simulink model "MMC_phase_hackathon_consensus_PWM_JABBAR_20260927"  (R2024b)
settings: Solver=FixedStepDiscrete  StartTime=t_init_sim  StopTime=sim_time  FixedStep=Ts  RelTol=1e-3
values from neighbouring files (symbols this model uses):
  a = 1    [script_MMC_phase_hackathon_consensus_PWM_JABBAR_20260927.m]
  C1low1_active = 1    [script_MMC_phase_hackathon_consensus_PWM_JABBAR_20260927.m]
  C2low1_active = 1    [script_MMC_phase_hackathon_consensus_PWM_JABBAR_20260927.m]
  C_bus = 4400e-6    (= 0.0044)    [script_MMC_phase_hackathon_consensus_PWM_JABBAR_20260927.m]
  C_M_extra = C_m-twist_high_side_C    [script_MMC_phase_hackathon_consensus_PWM_JABBAR_20260927.m]
  f0 = 50    [script_MMC_phase_hackathon_consensus_PWM_JABBAR_20260927.m]
  feeder_current_lower_rate_limit = -10    [script_MMC_phase_hackathon_consensus_PWM_JABBAR_20260927.m]    (also in twist_parameters.m = -500)
  feeder_current_tab = [0.328 0.217 0.162 0.132 0.109 0.094 0.083 0.075 0.068 0.062 0.058 0.054 ... (42 elements, 14x3)]    [feeder_current.mat]
  feeder_current_upper_rate_limit = 0.386/(20e-3)    (= 19.3)    [twist_parameters.m]
  is6VExternallySupplied = true    [script_MMC_phase_hackathon_consensus_PWM_JABBAR_20260927.m]
  isFeederJumperOpen = true    [script_MMC_phase_hackathon_consensus_PWM_JABBAR_20260927.m]
  L_arm = 100e-3    (= 0.1)    [script_MMC_phase_hackathon_consensus_PWM_JABBAR_20260927.m]
  m = 1    [script_MMC_phase_hackathon_consensus_PWM_JABBAR_20260927.m]
  power_losses = false    [script_MMC_phase_hackathon_consensus_PWM_JABBAR_20260927.m]
  R = 30    [script_MMC_phase_hackathon_consensus_PWM_JABBAR_20260927.m]
  R_arm = 0.2    [script_MMC_phase_hackathon_consensus_PWM_JABBAR_20260927.m]
  source_V = 0    [script_MMC_phase_hackathon_consensus_PWM_JABBAR_20260927.m]
  time_charge = 0.1    [script_MMC_phase_hackathon_consensus_PWM_JABBAR_20260927.m]
  time_decharge = 1.5    [script_MMC_phase_hackathon_consensus_PWM_JABBAR_20260927.m]
  Ts = 5e-7    (= 5e-07)    [script_MMC_phase_hackathon_consensus_PWM_JABBAR_20260927.m]
  twist_data_acquisition_delay = 50e-9    (= 5e-08)    [script_MMC_phase_hackathon_consensus_PWM_JABBAR_20260927.m]    (also in twist_parameters.m)
  twist_data_sampling_period = 1/twist_freq_data_sampling    (= 5e-05)    [script_MMC_phase_hackathon_consensus_PWM_JABBAR_20260927.m]    (also in twist_parameters.m)
  twist_dead_time = 200e-9    (= 2e-07)    [twist_parameters.m]
  twist_freq_switching = 200e3    (= 200000)    [twist_parameters.m]
  twist_high_side_adc_R = 1/(1/2e6 + 1/2e6 + 1/(330e3+5.6e3))    (= 251272.836178)    [twist_parameters.m]
  twist_high_side_C = 33e-6*4 + 4.7e-6*12    (= 0.0001884)    [twist_parameters.m]
  twist_high_side_feeder_R = 47e3+4.7e3    (= 51700)    [twist_parameters.m]
  twist_high_side_rC = 0.1    [twist_parameters.m]
  twist_low_side_adc_R = 150e3+470    (= 150470)    [twist_parameters.m]
  twist_low_side_C_ceramic = 3*4.7e-6    (= 1.41e-05)    [twist_parameters.m]
  twist_low_side_C_electrolytic = 47e-6    (= 4.7e-05)    [twist_parameters.m]
  twist_low_side_L = 33e-6    (= 3.3e-05)    [twist_parameters.m]
  twist_low_side_rC = 700e-3    (= 0.7)    [twist_parameters.m]
  twist_low_side_rL = 20e-3    (= 0.02)    [twist_parameters.m]
  twist_R_VCC = (tau_VCC/twist_high_side_C  - twist_high_side_rC)/(1-(tau_VCC/twist_high_side_C - twist_high_side_rC)/R_parallel)    (= 1110.74997822)    [twist_parameters.m]
  VDC = 48    [script_MMC_phase_hackathon_consensus_PWM_JABBAR_20260927.m]
undefined symbols (not defined in the file or in its folder): C_SM, feeder_current, gcbh, sps_rtmsupport, twist_low_side_lC
libraries: spsSeriesRLCBranchLib x135, spsTriangleGeneratorLib x60, spsMosfetLib x60, spsCurrentMeasurementLib x43, spsVoltageMeasurementLib x35, spsControlledCurrentSourceLib x30, spsDiodeLib x22, spsIdealSwitchLib x20, spsControlledVoltageSourceLib x1, spsGroundLib x1, spspowerguiLib x1
(part 1 of 19)
settings Model: Creator=ana  LastModifiedBy=ana

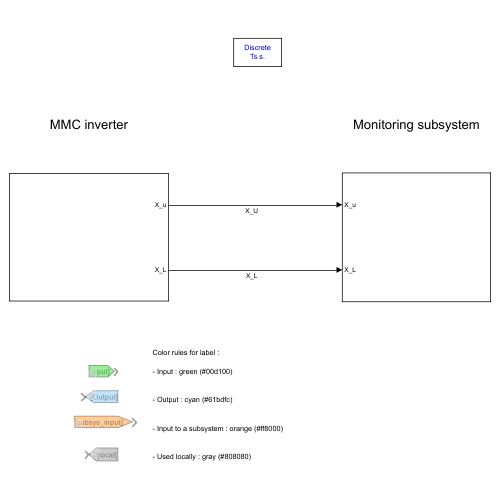
[thumbnail: Simulink's stored preview of the top-level diagram]
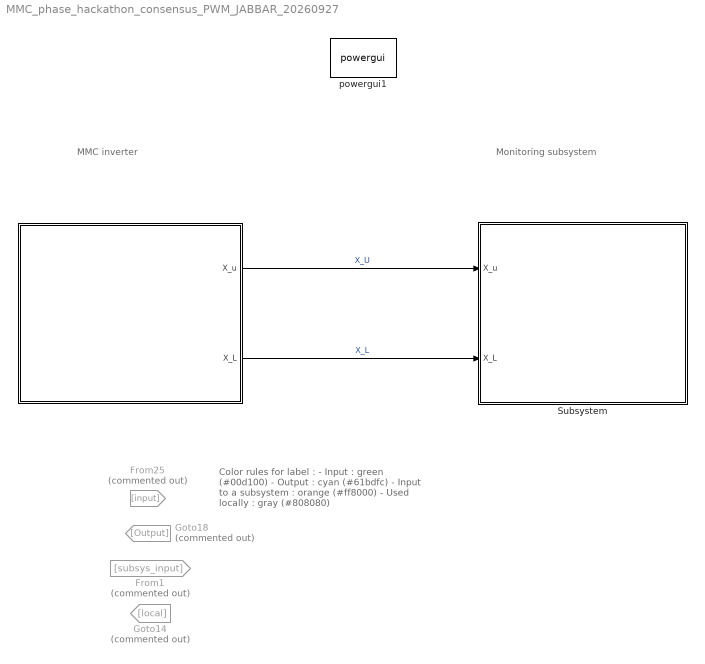
== system MMC_phase_hackathon_consensus_PWM_JABBAR_20260927 ==
  note: Color rules for label :
      |
      | - Input : green (#00d100)
      |
      |
      | - Output : cyan (#61bdfc)
      |
      |
      | - Input to a subsystem : orange (#ff8000)
      |
      |
      | - Used locally : gray (#808080)
  note: MMC inverter
  note: Monitoring subsystem
  " " : Subsystem
  From1 : From  Commented=on  GotoTag=subsys_input
  From25 : From  Commented=on  GotoTag=input
  Goto14 : Goto  Commented=on  GotoTag=local
  Goto18 : Goto  Commented=on  GotoTag=Output
  Subsystem : Subsystem
  powergui1 : spspowerguiLib/powergui  Priority=1  SimulationMode=Discrete  SampleTime=Ts  frequency=60  Iterations=50  frequencyindice=0  Pbase=100e6  ErrMax=1e-4  UnitsV=V  UnitsW=W  buscounter=0  FunctionMessages=off  echomessages=off  EnableUseOfTLC=off  CurrentSourceSwitches=off  DisableSnubberDevices=off  DisableRonSwitches=off  DisableVfSwitches=off  DisplayEquations=off  AutomaticDiscreteSolvers=off  SolverType=Backward Euler  Interpol=off  ExternalGateDelay=off  methode=off  Ts=0  x0status=blocks  SPID=off  SwTol=0  HookPort=off  NonlinearTolerance=1e-4  nMaxIteration=100  ContinueOnMaxIteration=off  RestoreLinks=warning  ResistiveCurrentMeasurement=off  Frange=[0:2:500]  Ylog=off  Xlog=on  ShowGrid=off  save=off  variable=ZData  structure=0  ZoomFFT=off  StartTime=0.0  cycles=1  DisplayStyle=1  fundamental=60  FreqAxis=off  MaxFrequency=1000  frequencyindicesteady=1  RmsSteady=1  display=off
  wires:
  " "/1(X_u) -> Subsystem/1(X_u)  "X_U"
  " "/2(X_L) -> Subsystem/2(X_L)  "X_L"

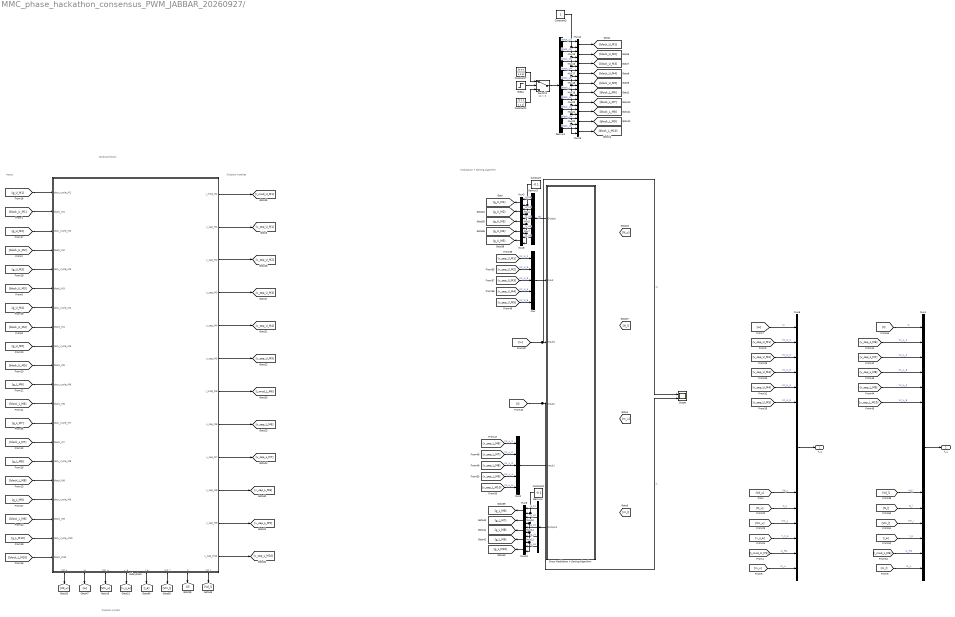
== system MMC_phase_hackathon_consensus_PWM_JABBAR_20260927/  ==
  note: Inputs
  note: Modulation + Sorting Algorithm
  note: Outputs modules
  note: Outputs system
  note: Hardware block
  Constant : Constant  Value=-0.1
  Constant1 : Constant  Value=-0.1
  Constant2 : Constant  Value=[1 1 1 1 1 1 1 1 1 1]
  Constant3 : Constant
  Constant7 : Constant  Value=[0 0 0 0 0 0 0 0 0 0]
  Demux1 : Demux  Outputs=10
  Demux3 : Demux  Outputs=5
  Demux4 : Demux  Outputs=5
  Mux : Mux  Inputs=5
  Mux1 : Mux  Inputs=17
  Mux{3..5,7..23} (20 alike) : Mux  Inputs=2
  Mux2 : Mux  Inputs=5
  Mux6 : Mux  Inputs=17
  Scope : Scope  NumInputPorts=2
  Sinus Modulation + Sorting Algorithm : Subsystem
      settings: PortSchema="{\"entries\":[{\"content\":{\"sides\":[{\"content\":{\"connectorIds\":[\"Out1\",\"In1\",\"In2\",\"In3\",\"In4\",\"Out2\"]},\"type\":\"ConnectorPlacement.EquallySpacedRectSide\",\"uuid\":\"ad8c3084-d308-4367-9563-bcedaf510cf0\"},{\"content\":{\"side\":\"RIGHT\"},\"type\":\"ConnectorPlacement.EquallySpacedRectSide\",\"uuid\":\"bc60d766-efa5-4acc-9a9d-e305ac7836ae\"},{\"content\":{\"side\":\"TOP\"},\"type\":\"ConnectorPlacement.EquallySpacedRectSide\",\"uuid\":\"8fba04a6-3f78-400c-9de2-20d6df686ca2\"}]},\"type\":\"ConnectorPlacement.EquallySpacedConnector\",\"uuid\":\"e4a9f561-cf27-428b-9d42-5aa201811d00\"}],\"packageUris\":[\"http://schema.mathworks.com/mf0/Connector/R2020b\"],\"version\":\"1.0\"}"
  Step1 : Step  Time=time_charge  SampleTime=Ts
  Subsystem : Subsystem
      settings: PortSchema="{\"entries\":[{\"content\":{\"sides\":[{\"content\":{\"connectorIds\":[\"In1\",\"In2\",\"In3\",\"In4\",\"In5\",\"In6\",\"In7\",\"In8\",\"In9\",\"In10\",\"In11\",\"In12\",\"In13\",\"In14\",\"In15\",\"In16\",\"In17\",\"In18\",\"In19\",\"In20\"]},\"type\":\"ConnectorPlacement.EquallySpacedRectSide\",\"uuid\":\"46d0b6b2-241e-4eaa-b5f4-7cb03ad6e4f0\"},{\"content\":{\"connectorIds\":[\"Out1\",\"Out2\",\"Out3\",\"Out4\",\"Out5\",\"Out6\",\"Out7\",\"Out8\",\"Out9\",\"Out10\",\"Out11\",\"Out12\"],\"side\":\"RIGHT\"},\"type\":\"ConnectorPlacement.EquallySpacedRectSide\",\"uuid\":\"f0391c40-5bbd-42ea-8549-0acba96c1793\"},{\"content\":{\"side\":\"TOP\"},\"type\":\"ConnectorPlacement.EquallySpacedRectSide\",\"uuid\":\"1ede63b4-6869-46b3-8b67-84e7db18bcff\"},{\"content\":{\"connectorIds\":[\"Out13\",\"Out14\",\"Out15\",\"Out16\",\"Out17\",\"Out18\",\"Out19\",\"Out20\"],\"side\":\"BOTTOM\"},\"type\":\"ConnectorPlacement.EquallySpacedRectSide\",\"uuid\":\"c0e3b199-6126-45b0-9783-8fc4162e2280\"}]},\"type\":\"ConnectorPlacement.EquallySpacedConnector\",\"uuid\":\"8bedc799-aa9e-49e4-9c41-8dbcca404e51\"}],\"packageUris\":[\"http://schema.mathworks.com/mf0/Connector/R2020b\"],\"version\":\"1.0\"}"
  Switch1 : Switch  Criteria=u2 > Threshold  SaturateOnIntegerOverflow=off  InputSameDT=off
  X_u : Outport
  X_L : Outport  Port=2
  wires:
  Mux6/1 -> X_u/1
  [iu] -> Mux6/1  "Iu"
  [Vd_u] -> Mux6/12  "Vd_u"
  ? -> [N_u]  "N_u"
  [N_u] -> Mux6/13  "N_u"
  [Vm_u] -> Mux6/14  "Vm_u"
  [v_s_a] -> Mux6/15  "V_s_a"
  Step1/1 -> Switch1/2
  Switch1/1 -> Demux1/1
  Constant7/1 -> Switch1/1
  Constant2/1 -> Switch1/3
  [i_mod_U_M1] -> Mux6/16  "Iu_M1"
  ? -> [N_l]  "N_l"
  [il] -> Mux1/1  "iL"
  Mux1/1 -> X_L/1
  [i_mod_L_M6] -> Mux1/16  "iL_M1"
  [Vd_l] -> Mux1/12  "Vd_l"
  [Vm_l] -> Mux1/14  "Vm_l"
  [N_l] -> Mux1/13  "N_l"
  [i_a] -> Mux1/15  "I_a"
  [v_cap_U_M1] -> Mux6/2  "Vc_U_1"
  [v_cap_U_M2] -> Mux6/3  "Vc_U_2"
  [v_cap_U_M3] -> Mux6/4  "Vc_U_3"
  [v_cap_U_M4] -> Mux6/5  "Vc_U_4"
  [v_cap_U_M5] -> Mux6/6  "Vc_U_5"
  ? -> Mux6/7  "Vm_U_1"
  ? -> Mux6/8  "Vm_U_2"
  ? -> Mux6/9  "Vm_U_3"
  ? -> Mux6/10  "Vm_U_4"
  ? -> Mux6/11  "Vm_U_5"
  [v_cap_L_M6] -> Mux1/2  "Vc_L_1"
  [v_cap_L_M7] -> Mux1/3  "Vc_L_2"
  [v_cap_L_M8] -> Mux1/4  "Vc_L_3"
  [v_cap_L_M9] -> Mux1/5  "Vc_L_4"
  [v_cap_L_M10] -> Mux1/6  "Vc_L_5"
  ? -> Mux1/7  "Vm_L_1"
  ? -> Mux1/8  "Vm_L_2"
  ? -> Mux1/9  "Vm_L_3"
  ? -> Mux1/10  "Vm_L_4"
  ? -> Mux1/11  "Vm_L_5"
  ? -> [m_u]  "m_u"
  ? -> [m_l]  "m_l"
  [m_u] -> Mux6/17  "m_u"
  [m_l] -> Mux1/17  "m_L"
  Sinus Modulation + Sorting Algorithm/1(Output) -> Demux3/1  "gU"
  Mux/1 -> Sinus Modulation + Sorting Algorithm/1(Input)
  [v_cap_U_M1] -> Mux/1  "Vc_U_1"
  [v_cap_U_M2] -> Mux/2  "Vc_U_2"
  [v_cap_U_M3] -> Mux/3  "Vc_U_3"
  [v_cap_U_M4] -> Mux/4  "Vc_U_4"
  [v_cap_U_M5] -> Mux/5  "Vc_U_5"
  [v_cap_L_M6] -> Mux2/1  "Vc_L_1"
  [v_cap_L_M7] -> Mux2/2  "Vc_L_2"
  [v_cap_L_M8] -> Mux2/3  "Vc_L_3"
  [v_cap_L_M9] -> Mux2/4  "Vc_L_4"
  [v_cap_L_M10] -> Mux2/5  "Vc_L_5"
  Mux3/1 -> [g_U_M1]
  Mux8/1 -> [g_U_M5]
  Mux7/1 -> [g_U_M4]
  Mux5/1 -> [g_U_M3]
  Mux4/1 -> [g_U_M2]
  Demux3/1 -> Mux3/1  "g_U1"
  Demux3/2 -> Mux4/1  "g_U2"
  Demux3/3 -> Mux5/1  "g_U3"
  Demux3/4 -> Mux7/1  "g_U4"
  Demux3/5 -> Mux8/1  "g_U5"
  Constant/1 -> Mux8/2, Mux7/2, Mux5/2, Mux4/2, Mux3/2
  Constant1/1 -> Mux13/2, Mux12/2, Mux11/2, Mux10/2, Mux9/2
  Mux9/1 -> [g_L_M6]
  Mux10/1 -> [g_L_M7]
  Mux11/1 -> [g_L_M8]
  Mux12/1 -> [g_L_M9]
  Mux13/1 -> [g_L_M10]
  Demux4/1 -> Mux9/1  "g_L1"
  Demux4/2 -> Mux10/1  "g_L2"
  Demux4/3 -> Mux11/1  "g_L3"
  Demux4/4 -> Mux12/1  "g_L4"
  Demux4/5 -> Mux13/1  "g_L5"
  Demux1/1 -> Mux14/1  "block_U1"
  Constant3/1 -> Mux23/2, Mux22/2, Mux21/2, Mux20/2, Mux19/2, Mux18/2, Mux17/2, Mux16/2, Mux15/2, Mux14/2
  Demux1/2 -> Mux15/1  "block_U2"
  Demux1/3 -> Mux16/1  "block_U3"
  Demux1/4 -> Mux17/1  "block_U4"
  Demux1/5 -> Mux18/1  "block_U5"
  Demux1/6 -> Mux19/1  "block_L1"
  Demux1/7 -> Mux20/1  "block_L2"
  Demux1/8 -> Mux21/1  "block_L3"
  Demux1/9 -> Mux22/1  "block_L4"
  Demux1/10 -> Mux23/1  "block_L5"
  Mux14/1 -> [block_U_M1]
  Mux15/1 -> [block_U_M2]
  Mux16/1 -> [block_U_M3]
  Mux18/1 -> [block_U_M5]
  Mux17/1 -> [block_U_M4]
  Mux19/1 -> [block_L_M6]
  Mux20/1 -> [block_L_M7]
  Mux21/1 -> [block_L_M8]
  Mux22/1 -> [block_L_M9]
  Mux23/1 -> [block_L_M10]
  [g_U_M1] -> Subsystem/1(duty_cycle_M1)
  [block_U_M1] -> Subsystem/2(block_M1)
  [g_U_M2] -> Subsystem/3(duty_cycle_M2)
  [block_U_M2] -> Subsystem/4(block_M2)
  [g_U_M3] -> Subsystem/5(duty_cycle_M3)
  [block_U_M3] -> Subsystem/6(block_M3)
  [g_U_M4] -> Subsystem/7(duty_cycle_M4)
  [block_U_M4] -> Subsystem/8(block_M4)
  [g_U_M5] -> Subsystem/9(duty_cycle_M5)
  [block_U_M5] -> Subsystem/10(block_M5)
  [g_L_M6] -> Subsystem/11(duty_cycle_M6)
  [block_L_M6] -> Subsystem/12(block_M6)
  [g_L_M7] -> Subsystem/13(duty_cycle_M7)
  [block_L_M7] -> Subsystem/14(block_M7)
  [g_L_M8] -> Subsystem/15(duty_cycle_M8)
  [block_L_M8] -> Subsystem/16(block_M8)
  [g_L_M9] -> Subsystem/17(duty_cycle_M9)
  [block_L_M9] -> Subsystem/18(block_M9)
  [g_L_M10] -> Subsystem/19(duty_cycle_M10)
  [block_L_M10] -> Subsystem/20(block_M10)
  Subsystem/1(i_mod_M1) -> [i_mod_U_M1]
  Subsystem/2(v_cap_M1) -> [v_cap_U_M1]
  Subsystem/3(v_cap_M2) -> [v_cap_U_M2]
  Subsystem/4(v_cap_M3) -> [v_cap_U_M3]
  Subsystem/5(v_cap_M4) -> [v_cap_U_M4]
  Subsystem/6(v_cap_M5) -> [v_cap_U_M5]
  Subsystem/7(i_mod_M6) -> [i_mod_L_M6]
  Subsystem/8(v_cap_M6) -> [v_cap_L_M6]
  Subsystem/9(v_cap_M7) -> [v_cap_L_M7]
  Subsystem/10(v_cap_M8) -> [v_cap_L_M8]
  Subsystem/11(v_cap_M9) -> [v_cap_L_M9]
  Subsystem/12(v_cap_M10) -> [v_cap_L_M10]
  Subsystem/16(v_a) -> [v_s_a]
  Subsystem/20(Vd_l) -> [Vd_l]
  Subsystem/19(il) -> [il]
  Subsystem/15(Vm_u) -> [Vm_u]
  Subsystem/14(iu) -> [iu]
  Subsystem/13(Vd_u) -> [Vd_u]
  Subsystem/17(i_a) -> [i_a]
  Subsystem/18(Vm_l) -> [Vm_l]
  Sinus Modulation + Sorting Algorithm/2(Output1) -> Demux4/1
  [il] -> Scope/2, Sinus Modulation + Sorting Algorithm/3(Input2)  "iL"
  [iu] -> Scope/1, Sinus Modulation + Sorting Algorithm/2(Input3)  "Iu"
  Mux2/1 -> Sinus Modulation + Sorting Algorithm/4(Input1)

== system MMC_phase_hackathon_consensus_PWM_JABBAR_20260927/Subsystem ==
  note: To workspace
  X_u : Inport
  X_L : Inport  Port=2
  Constant : Constant  Value=2
  Demux : Demux  Outputs=2
  Demux{1..4} (4 alike) : Demux  Outputs=17
  Divide : Product  Inputs=*/
  Mux : Mux  Inputs=5
  Mux{1..3,8} (4 alike) : Mux  Inputs=2
  Mux5 : Mux  Inputs=5
  Scope{,1..2,4..5} (5 alike) : Scope
  Scope3 : Scope  NumInputPorts=7
  Sum : Sum  Inputs=|++
  To Workspace1 : ToWorkspace  VariableName=vm_1  SaveFormat=Structure With Time  SampleTime=-1
  To Workspace10 : ToWorkspace  VariableName=vc_1  SaveFormat=Structure With Time  SampleTime=-1
  To Workspace11 : ToWorkspace  VariableName=va  SaveFormat=Structure With Time  SampleTime=-1
  To Workspace12 : ToWorkspace  VariableName=m_u  SaveFormat=Structure With Time  SampleTime=-1
  To Workspace13 : ToWorkspace  VariableName=i_u_M1_meas  SaveFormat=Structure With Time  SampleTime=-1
  To Workspace14 : ToWorkspace  VariableName=vm_10  SaveFormat=Structure With Time  SampleTime=-1
  To Workspace15 : ToWorkspace  VariableName=vm_2  SaveFormat=Structure With Time  SampleTime=-1
  To Workspace16 : ToWorkspace  VariableName=vm_3  SaveFormat=Structure With Time  SampleTime=-1
  To Workspace17 : ToWorkspace  VariableName=vm_4  SaveFormat=Structure With Time  SampleTime=-1
  To Workspace18 : ToWorkspace  VariableName=vm_5  SaveFormat=Structure With Time  SampleTime=-1
  To Workspace19 : ToWorkspace  VariableName=vc_10  SaveFormat=Structure With Time  SampleTime=-1
  To Workspace2 : ToWorkspace  VariableName=vc_2  SaveFormat=Structure With Time  SampleTime=-1
  To Workspace20 : ToWorkspace  VariableName=ia  SaveFormat=Structure With Time  SampleTime=-1
  To Workspace21 : ToWorkspace  VariableName=m_l  SaveFormat=Structure With Time  SampleTime=-1
  To Workspace22 : ToWorkspace  VariableName=i_l_M1_meas  SaveFormat=Structure With Time  SampleTime=-1
  To Workspace23 : ToWorkspace  VariableName=vm_6  SaveFormat=Structure With Time  SampleTime=-1
  To Workspace24 : ToWorkspace  VariableName=vm_7  SaveFormat=Structure With Time  SampleTime=-1
  To Workspace25 : ToWorkspace  VariableName=vm_8  SaveFormat=Structure With Time  SampleTime=-1
  To Workspace26 : ToWorkspace  VariableName=vm_9  SaveFormat=Structure With Time  SampleTime=-1
  To Workspace27 : ToWorkspace  VariableName=vc_6  SaveFormat=Structure With Time  SampleTime=-1
  To Workspace28 : ToWorkspace  VariableName=vc_7  SaveFormat=Structure With Time  SampleTime=-1
  To Workspace29 : ToWorkspace  VariableName=vc_8  SaveFormat=Structure With Time  SampleTime=-1
  To Workspace3 : ToWorkspace  VariableName=vc_3  SaveFormat=Structure With Time  SampleTime=-1
  To Workspace30 : ToWorkspace  VariableName=vc_9  SaveFormat=Structure With Time  SampleTime=-1
  To Workspace31 : ToWorkspace  VariableName=vd_l  SaveFormat=Structure With Time  SampleTime=-1
  To Workspace32 : ToWorkspace  VariableName=N_l  SaveFormat=Structure With Time  SampleTime=-1
  To Workspace33 : ToWorkspace  VariableName=i_l  SaveFormat=Structure With Time  SampleTime=-1
  To Workspace34 : ToWorkspace  VariableName=vm_l  SaveFormat=Structure With Time  SampleTime=-1
  To Workspace4 : ToWorkspace  VariableName=vc_4  SaveFormat=Structure With Time  SampleTime=-1
  To Workspace5 : ToWorkspace  VariableName=vc_5  SaveFormat=Structure With Time  SampleTime=-1
  To Workspace6 : ToWorkspace  VariableName=vd_u  SaveFormat=Structure With Time  SampleTime=-1
  To Workspace7 : ToWorkspace  VariableName=N_u  SaveFormat=Structure With Time  SampleTime=-1
  To Workspace8 : ToWorkspace  VariableName=i_u  SaveFormat=Structure With Time  SampleTime=-1
  To Workspace9 : ToWorkspace  VariableName=vm_u  SaveFormat=Structure With Time  SampleTime=-1
  wires:
  Demux4/15 -> To Workspace20/1  "i_a"
  Demux1/4 -> To Workspace3/1  "Vc_3"
  Demux4/17 -> To Workspace21/1  "m_l"
  X_L/1 -> Demux3/1, [l_SW]
  Demux2/14 -> [v_m_u]  "Vm_u"
  Demux1/2 -> To Workspace10/1  "Vc_1"
  Demux1/14 -> To Workspace9/1  "Vm_u"
  Mux2/1 -> Scope3/2  "V_m_U/L"
  Demux4/3 -> To Workspace28/1  "Vc_2"
  Demux1/7 -> To Workspace1/1  "Vm_1"
  Demux4/1 -> To Workspace33/1  "i_l"
  Demux2/1 -> Mux3/1  "i_u"
  Demux2/4 -> Mux/3  "V_uc_3"
  [v_m_u] -> Mux2/1
  [i_a] -> Scope3/7  "I_a"
  X_u/1 -> Demux2/1, [u_SW]
  Demux2/15 -> [v_a]  "V_a"
  Demux3/6 -> Mux5/5  "Vc_l_5"
  Demux2/16 -> Mux3/2  "iu_M1_meas"
  [i_l] -> Sum/2
  Demux3/1 -> Mux8/1  "i_l"
  Demux4/7 -> To Workspace23/1  "Vm_1"
  Demux1/11 -> To Workspace18/1  "Vm_5"
  Demux3/16 -> Mux8/2  "il_M1_meas"
  Demux1/13 -> To Workspace7/1  "N_u"
  Demux4/9 -> To Workspace25/1  "Vm_3"
  Demux2/3 -> Mux/2  "Vc_u_2"
  [i_u] -> Mux1/1
  Demux4/11 -> To Workspace14/1  "Vm_5"
  Mux5/1 -> [v_c_l]
  Demux4/8 -> To Workspace24/1  "Vm_2"
  [l_SW] -> Demux4/1  "L_SW"
  Demux1/5 -> To Workspace4/1  "Vc_4"
  Mux8/1 -> [i_l]
  Mux3/1 -> [i_u]  "I_u"
  Demux3/3 -> Mux5/2  "Vc_l_2"
  Constant/1 -> Divide/2
  Demux3/5 -> Mux5/4  "Vc_l_4"
  Demux4/4 -> To Workspace29/1  "Vc_3"
  Sum/1 -> Scope1/1, Divide/1  "I_u + I_L"
  Demux3/15 -> [i_a]  "i_a"
  Divide/1 -> Scope/1, Demux/1  "(I_U + I_L)/2"
  Demux1/3 -> To Workspace2/1  "Vc_2"
  Demux3/2 -> Mux5/1  "Vc_l_1"
  Demux1/16 -> To Workspace13/1  "iu_M1_meas"
  Demux2/5 -> Mux/4  "Vc_u_4"
  [v_a] -> Scope5/1, Scope3/3  "V_a"
  Demux4/16 -> To Workspace22/1  "il_M1_meas"
  Demux1/10 -> To Workspace17/1  "Vm_4"
  [i_l] -> Mux1/2
  [u_SW] -> Demux1/1  "u_SW"
  Demux1/17 -> To Workspace12/1  "m_u"
  Demux1/15 -> To Workspace11/1  "Va"
  Demux1/12 -> To Workspace6/1  "Vd_u"
  Demux2/2 -> Mux/1  "Vc_u_1"
  Demux4/13 -> To Workspace32/1  "N_l"
  Demux1/9 -> To Workspace16/1  "Vm_3"
  Demux4/6 -> To Workspace19/1  "Vc_5"
  Demux4/2 -> To Workspace27/1  "Vc_1"
  Demux4/14 -> To Workspace34/1  "Vm_l"
  Demux/1 -> [i_Sigma_a]
  [v_c_l] -> Scope2/1, Scope3/5  "V_c_L"
  Demux2/6 -> Mux/5  "Vc_u_5"
  Demux1/8 -> To Workspace15/1  "Vm_2"
  [v_c_u] -> Scope4/1, Scope3/1  "V_c_u"
  Demux1/6 -> To Workspace5/1  "Vc_5"
  Demux1/1 -> To Workspace8/1  "i_u"
  [v_m_l] -> Mux2/2
  [i_u] -> Sum/1
  [i_Sigma_a] -> Scope3/4  "i_Sigma"
  Demux4/12 -> To Workspace31/1  "Vd_l"
  Demux3/14 -> [v_m_l]  "Vm_l"
  Mux1/1 -> Scope3/6  "I_U/L"
  Demux3/4 -> Mux5/3  "Vc_l_3"
  Mux/1 -> [v_c_u]  "V_c_u"
  Demux4/10 -> To Workspace26/1  "Vm_4"
  Demux4/5 -> To Workspace30/1  "Vc_4"

== system MMC_phase_hackathon_consensus_PWM_JABBAR_20260927/ /Sinus Modulation + Sorting Algorithm ==
  note: Modulation reference
  Input : Inport
  Input3 : Inport  Port=2
  Input2 : Inport  Port=3
  Input1 : Inport  Port=4
  Constant4 : Constant  Value=a*1/2
  Gain1 : Gain  Gain=m*1/2
  Sine Wave : Sin  Frequency=2*pi*f0  SampleTime=Ts
  Subsystem1 : Subsystem
  Subsystem2 : Subsystem
  Sum1 : Sum  Inputs=|+-
  Sum2 : Sum  Inputs=|++
  Output : Outport
  Output1 : Outport  Port=2
  tag scope: Nl_a=global, Nu_a=global
  wires:
  Constant4/1 -> Sum2/1, Sum1/1
  Sine Wave/1 -> Gain1/1
  Gain1/1 -> Sum1/2, Sum2/2
  Sum1/1 -> [Nu_a]
  Sum2/1 -> [Nl_a]
  Subsystem1/1(Out1) -> Output/1
  Input/1 -> Subsystem1/1(Input)
  Subsystem2/1(Output) -> Output1/1
  Input1/1 -> Subsystem2/1(Input)
  Input2/1 -> Subsystem2/2(Input1)
  Input3/1 -> Subsystem1/2(Input1)

== system MMC_phase_hackathon_consensus_PWM_JABBAR_20260927/ /Subsystem ==
  note: MMC electrical circuit connected to the modules hardware block
  duty_cycle_M1 : Inport
  block_M1 : Inport  Port=2
  duty_cycle_M2 : Inport  Port=3
  block_M2 : Inport  Port=4
  duty_cycle_M3 : Inport  Port=5
  block_M3 : Inport  Port=6
  duty_cycle_M4 : Inport  Port=7
  block_M4 : Inport  Port=8
  duty_cycle_M5 : Inport  Port=9
  block_M5 : Inport  Port=10
  duty_cycle_M6 : Inport  Port=11
  block_M6 : Inport  Port=12
  duty_cycle_M7 : Inport  Port=13
  block_M7 : Inport  Port=14
  duty_cycle_M8 : Inport  Port=15
  block_M8 : Inport  Port=16
  duty_cycle_M9 : Inport  Port=17
  block_M9 : Inport  Port=18
  duty_cycle_M10 : Inport  Port=19
  block_M10 : Inport  Port=20
  AC Load1 : spsSeriesRLCBranchLib/Series RLC Branch  LConnTagsString=__new0  RConnTagsString=__new0  BranchType=RL  Resistance=R_arm  Inductance=L_arm  SetiL0=off  InitialCurrent=0  Capacitance=C_SM  Setx0=off  InitialVoltage=0  Measurements=None
  AC Load2 : spsSeriesRLCBranchLib/Series RLC Branch  LConnTagsString=__new0  RConnTagsString=__new0  BranchType=RL  Resistance=R_arm  Inductance=L_arm  SetiL0=off  InitialCurrent=0  Capacitance=C_SM  Setx0=off  InitialVoltage=0  Measurements=None
  AC Load3 : spsSeriesRLCBranchLib/Series RLC Branch  LConnTagsString=__new0  RConnTagsString=__new0  BranchType=R  Resistance=R  Inductance=L_arm  SetiL0=off  InitialCurrent=0  Capacitance=C_SM  Setx0=off  InitialVoltage=0  Measurements=None
  AC Load4 : spsSeriesRLCBranchLib/Series RLC Branch  LConnTagsString=__new0  RConnTagsString=__new0  BranchType=C  Resistance=R  Inductance=L_arm  SetiL0=off  InitialCurrent=0  Capacitance=C_bus  Setx0=off  InitialVoltage=0  Measurements=None
  AC Load5 : spsSeriesRLCBranchLib/Series RLC Branch  LConnTagsString=__new0  RConnTagsString=__new0  BranchType=C  Resistance=R  Inductance=L_arm  SetiL0=off  InitialCurrent=0  Capacitance=C_bus  Setx0=off  InitialVoltage=0  Measurements=None
  Controlled Voltage Source : spsControlledVoltageSourceLib/Controlled Voltage Source  Initialize=on  Source_Type=DC  Amplitude=0  Phase=0  Frequency=0  Measurements=None
  Current Measurement1 : spsCurrentMeasurementLib/Current Measurement  PhasorSimulation=off  OutputType=Complex  PSBequivalent=0
  Current Measurement2 : spsCurrentMeasurementLib/Current Measurement  PhasorSimulation=off  OutputType=Complex  PSBequivalent=0
  Current Measurement4 : spsCurrentMeasurementLib/Current Measurement  PhasorSimulation=off  OutputType=Complex  PSBequivalent=0
  Diode1 : spsDiodeLib/Diode  Ron=0.001  Lon=0  Vf=0.8  IC=0  UseSnubber=0  Rs=1e5  Cs=inf  Measurements=off
  Diode2 : spsDiodeLib/Diode  Ron=0.001  Lon=0  Vf=0.8  IC=0  UseSnubber=0  Rs=1e5  Cs=inf  Measurements=off
  Ground : spsGroundLib/Ground  LConnTagsString=a
  Step2 : Step  Time=time_decharge  Before=VDC  After=0  SampleTime=0
  Subsystem : Subsystem
      settings: PortSchema="{\"entries\":[{\"content\":{\"sides\":[{\"content\":{\"connectorIds\":[\"LConn1\",\"In1\",\"In2\",\"In3\",\"In4\",\"In5\",\"In6\",\"In7\",\"In8\",\"In9\",\"In10\",\"LConn2\"]},\"type\":\"ConnectorPlacement.EquallySpacedRectSide\",\"uuid\":\"af96ca56-9fdb-47ea-8e31-50f481daafc4\"},{\"content\":{\"connectorIds\":[\"Out1\",\"Out2\",\"Out3\",\"Out4\",\"Out5\",\"Out6\"],\"side\":\"RIGHT\"},\"type\":\"ConnectorPlacement.EquallySpacedRectSide\",\"uuid\":\"66f6256f-049a-4c8a-aad5-8d93b148b037\"},{\"content\":{\"side\":\"TOP\"},\"type\":\"ConnectorPlacement.EquallySpacedRectSide\",\"uuid\":\"596eb3e1-7761-4783-802e-d9df31b3a9c1\"}]},\"type\":\"ConnectorPlacement.EquallySpacedConnector\",\"uuid\":\"34c6ade5-a2f4-48d8-9a9b-6856a5a88d76\"}],\"packageUris\":[\"http://schema.mathworks.com/mf0/Connector/R2020b\"],\"version\":\"1.0\"}"
  Subsystem1 : Subsystem
      settings: PortSchema="{\"entries\":[{\"content\":{\"sides\":[{\"content\":{\"connectorIds\":[\"LConn1\",\"In1\",\"In2\",\"In3\",\"In4\",\"In5\",\"In6\",\"In7\",\"In8\",\"In9\",\"In10\",\"LConn2\"]},\"type\":\"ConnectorPlacement.EquallySpacedRectSide\",\"uuid\":\"af96ca56-9fdb-47ea-8e31-50f481daafc4\"},{\"content\":{\"connectorIds\":[\"Out1\",\"Out2\",\"Out3\",\"Out4\",\"Out5\",\"Out6\"],\"side\":\"RIGHT\"},\"type\":\"ConnectorPlacement.EquallySpacedRectSide\",\"uuid\":\"66f6256f-049a-4c8a-aad5-8d93b148b037\"},{\"content\":{\"side\":\"TOP\"},\"type\":\"ConnectorPlacement.EquallySpacedRectSide\",\"uuid\":\"596eb3e1-7761-4783-802e-d9df31b3a9c1\"}]},\"type\":\"ConnectorPlacement.EquallySpacedConnector\",\"uuid\":\"34c6ade5-a2f4-48d8-9a9b-6856a5a88d76\"}],\"packageUris\":[\"http://schema.mathworks.com/mf0/Connector/R2020b\"],\"version\":\"1.0\"}"
  Voltage Measurement{5..8,14} (5 alike) : spsVoltageMeasurementLib/Voltage Measurement  PhasorSimulation=off  OutputType=Complex  PSBequivalent=0
  i_mod_M1 : Outport
  v_cap_M1 : Outport  Port=2
  v_cap_M2 : Outport  Port=3
  v_cap_M3 : Outport  Port=4
  v_cap_M4 : Outport  Port=5
  v_cap_M5 : Outport  Port=6
  i_mod_M6 : Outport  Port=7
  v_cap_M6 : Outport  Port=8
  v_cap_M7 : Outport  Port=9
  v_cap_M8 : Outport  Port=10
  v_cap_M9 : Outport  Port=11
  v_cap_M10 : Outport  Port=12
  Vd_u : Outport  Port=13
  iu : Outport  Port=14
  Vm_u : Outport  Port=15
  v_a : Outport  Port=16
  i_a : Outport  Port=17
  Vm_l : Outport  Port=18
  il : Outport  Port=19
  Vd_l : Outport  Port=20
  wires:
  Voltage Measurement7/1 -> Vd_u/1
  Current Measurement2/1 -> i_a/1
  Step2/1 -> Controlled Voltage Source/1
  Voltage Measurement5/1 -> Vm_u/1
  Voltage Measurement6/1 -> v_a/1
  Voltage Measurement14/1 -> Vm_l/1
  duty_cycle_M1/1 -> Subsystem/1(duty_cycle_M1)
  block_M1/1 -> Subsystem/2(block_M1)
  duty_cycle_M2/1 -> Subsystem/3(duty_cycle_M2)
  block_M2/1 -> Subsystem/4(block_M2)
  duty_cycle_M3/1 -> Subsystem/5(duty_cycle_M3)
  block_M3/1 -> Subsystem/6(block_M3)
  duty_cycle_M4/1 -> Subsystem/7(duty_cycle_M4)
  block_M4/1 -> Subsystem/8(block_M4)
  duty_cycle_M5/1 -> Subsystem/9(duty_cycle_M5)
  block_M5/1 -> Subsystem/10(block_M5)
  Subsystem/1(i_mod_M1) -> i_mod_M1/1
  Subsystem/6(v_cap_M5) -> v_cap_M5/1
  Subsystem/5(v_cap_M4) -> v_cap_M4/1
  Subsystem/2(v_cap_M1) -> v_cap_M1/1
  Subsystem/3(v_cap_M2) -> v_cap_M2/1
  Subsystem/4(v_cap_M3) -> v_cap_M3/1
  block_M9/1 -> Subsystem1/8(block_M4)
  duty_cycle_M9/1 -> Subsystem1/7(duty_cycle_M4)
  block_M10/1 -> Subsystem1/10(block_M5)
  duty_cycle_M10/1 -> Subsystem1/9(duty_cycle_M5)
  duty_cycle_M6/1 -> Subsystem1/1(duty_cycle_M1)
  duty_cycle_M7/1 -> Subsystem1/3(duty_cycle_M2)
  block_M7/1 -> Subsystem1/4(block_M2)
  duty_cycle_M8/1 -> Subsystem1/5(duty_cycle_M3)
  block_M6/1 -> Subsystem1/2(block_M1)
  block_M8/1 -> Subsystem1/6(block_M3)
  Subsystem1/1(i_mod_M1) -> i_mod_M6/1
  Subsystem1/2(v_cap_M1) -> v_cap_M6/1
  Subsystem1/3(v_cap_M2) -> v_cap_M7/1
  Subsystem1/4(v_cap_M3) -> v_cap_M8/1
  Subsystem1/5(v_cap_M4) -> v_cap_M9/1
  Subsystem1/6(v_cap_M5) -> v_cap_M10/1
  Current Measurement4/1 -> iu/1
  Voltage Measurement8/1 -> Vd_l/1
  Current Measurement1/1 -> il/1
  connections:
  Controlled Voltage Source/LConn1 -- Voltage Measurement8/LConn2 -- Diode1/RConn1
  AC Load2/LConn1 -- AC Load4/LConn1 -- Diode2/RConn1 -- Voltage Measurement7/LConn2
  Current Measurement4/RConn1 -- Voltage Measurement5/LConn1 -- Subsystem/LConn1
  Voltage Measurement14/LConn2 -- Subsystem1/LConn2 -- Current Measurement1/LConn1
  AC Load2/RConn1 -- Current Measurement4/LConn1
  Voltage Measurement6/LConn1 -- Subsystem1/LConn1 -- Voltage Measurement14/LConn1 -- Voltage Measurement5/LConn2 -- Subsystem/LConn2 -- AC Load3/RConn1
  Ground/LConn1 -- AC Load5/LConn1 -- AC Load4/RConn1 -- Current Measurement2/RConn1
  AC Load1/RConn1 -- Current Measurement1/RConn1
  Voltage Measurement7/LConn1 -- Controlled Voltage Source/RConn1 -- Diode2/LConn1
  AC Load1/LConn1 -- Diode1/LConn1 -- Voltage Measurement8/LConn1 -- AC Load5/RConn1
  Current Measurement2/LConn1 -- Voltage Measurement6/LConn2 -- AC Load3/LConn1

== system MMC_phase_hackathon_consensus_PWM_JABBAR_20260927/ /Sinus Modulation + Sorting Algorithm/Subsystem1 ==
  Input : Inport
  Input1 : Inport  Port=2
  Constant : Constant  OutDataTypeStr=single
  Constant1 : Constant  Value=2  OutDataTypeStr=single
  Constant2 : Constant  Value=3  OutDataTypeStr=single
  Constant3 : Constant  Value=4  OutDataTypeStr=single
  Constant4 : Constant  Value=5  OutDataTypeStr=single
  Mux : Mux  Inputs=5
  Subsystem : Subsystem
  Subsystem1 : Subsystem
  Subsystem2 : Subsystem
  Subsystem3 : Subsystem
  Subsystem4 : Subsystem
  Out1 : Outport
  tag scope: s1=global, s2U=global, s3U=global, s4U=global, s5U=global
  wires:
  Constant/1 -> Subsystem/1(sm_id)
  Subsystem/1(gate_signal) -> Mux/1, [s1]
  Subsystem1/1(gate_signal) -> Mux/2, [s2U]
  Constant1/1 -> Subsystem1/1(sm_id)
  Constant2/1 -> Subsystem2/1(sm_id)
  Subsystem2/1(gate_signal) -> Mux/3, [s3U]
  Constant3/1 -> Subsystem3/1(sm_id)
  Constant4/1 -> Subsystem4/1(sm_id)
  Subsystem4/1(gate_signal) -> Mux/5, [s5U]
  Input/1 -> Subsystem4/2(Vc_am), Subsystem3/2(Vc_am), Subsystem2/2(Vc_am), Subsystem1/2(Vc_am), Subsystem/2(Vc_am)
  Subsystem3/1(gate_signal) -> Mux/4, [s4U]
  Mux/1 -> Out1/1
  Input1/1 -> Subsystem/3(Input), Subsystem4/3(Input), Subsystem3/3(Input), Subsystem2/3(Input), Subsystem1/3(Input)

== system MMC_phase_hackathon_consensus_PWM_JABBAR_20260927/ /Sinus Modulation + Sorting Algorithm/Subsystem2 ==
  Input : Inport
  Input1 : Inport  Port=2
  Constant : Constant  OutDataTypeStr=double
  Constant1 : Constant  Value=2  OutDataTypeStr=double
  Constant2 : Constant  Value=3  OutDataTypeStr=double
  Constant3 : Constant  Value=4  OutDataTypeStr=double
  Constant4 : Constant  Value=5  OutDataTypeStr=double
  Mux : Mux  Inputs=5
  Subsystem : Subsystem
  Subsystem1 : Subsystem
  Subsystem2 : Subsystem
  Subsystem3 : Subsystem
  Subsystem4 : Subsystem
  Output : Outport
  tag scope: S5L=global, s1L=global, s2=global, s3=global, s4=global
  wires:
  Input/1 -> Subsystem/2(Vc_am), Subsystem2/2(Vc_am), Subsystem4/2(Vc_am), Subsystem3/2(Vc_am), Subsystem1/2(Vc_am)
  Subsystem4/1(gate_signal) -> Mux/5, [S5L]
  Constant4/1 -> Subsystem4/1(sm_id)
  Subsystem3/1(gate_signal) -> Mux/4, [s4]
  Constant3/1 -> Subsystem3/1(sm_id)
  Constant2/1 -> Subsystem2/1(sm_id)
  Constant1/1 -> Subsystem1/1(sm_id)
  Subsystem1/1(gate_signal) -> Mux/2, [s2]
  Subsystem/1(gate_signal) -> Mux/1, [s1L]
  Constant/1 -> Subsystem/1(sm_id)
  Subsystem2/1(gate_signal) -> Mux/3, [s3]
  Input1/1 -> Subsystem1/3(Input), Subsystem4/3(Input), Subsystem3/3(Input), Subsystem2/3(Input), Subsystem/3(Input)
  Mux/1 -> Output/1

== system MMC_phase_hackathon_consensus_PWM_JABBAR_20260927/ /Subsystem/Subsystem ==
  note: MMC electrical circuit connected to the modules hardware block
  note: MMC electrical circuit connected to the modules hardware block
  note: MMC electrical circuit connected to the modules hardware block
  note: MMC electrical circuit connected to the modules hardware block
  note: MMC electrical circuit connected to the modules hardware block
  duty_cycle_M1 : Inport
  block_M1 : Inport  Port=2
  duty_cycle_M2 : Inport  Port=3
  block_M2 : Inport  Port=4
  duty_cycle_M3 : Inport  Port=5
  block_M3 : Inport  Port=6
  duty_cycle_M4 : Inport  Port=7
  block_M4 : Inport  Port=8
  duty_cycle_M5 : Inport  Port=9
  block_M5 : Inport  Port=10
  AC Load{6..10} (5 alike) : spsSeriesRLCBranchLib/Series RLC Branch  LConnTagsString=__new0  RConnTagsString=__new0  BranchType=C  Resistance=R  Inductance=L_arm  SetiL0=off  InitialCurrent=0  Capacitance=C_M_extra  Setx0=on  InitialVoltage=source_V  Measurements=None
  Hardware M1 : Subsystem
  Hardware M2 : Subsystem
  Hardware M3 : Subsystem
  Hardware M4 : Subsystem
  Hardware M5 : Subsystem
  V1low_M1 : PMIOPort  Side=Left
  Low_GND_M5 : PMIOPort  Port=2  Side=Left
  i_mod_M1 : Outport
  v_cap_M1 : Outport  Port=2
  v_cap_M2 : Outport  Port=3
  v_cap_M3 : Outport  Port=4
  v_cap_M4 : Outport  Port=5
  v_cap_M5 : Outport  Port=6
  wires:
  Hardware M1/1(v_cap) -> v_cap_M1/1
  duty_cycle_M1/1 -> Hardware M1/1(duty_cycle)
  duty_cycle_M2/1 -> Hardware M2/1(duty_cycle)
  block_M5/1 -> Hardware M5/2(block)
  Hardware M3/1(v_cap) -> v_cap_M3/1
  block_M1/1 -> Hardware M1/2(block)
  Hardware M1/2(i_mod) -> i_mod_M1/1
  duty_cycle_M4/1 -> Hardware M4/1(duty_cycle)
  block_M2/1 -> Hardware M2/2(block)
  Hardware M5/1(v_cap) -> v_cap_M5/1
  Hardware M2/1(v_cap) -> v_cap_M2/1
  duty_cycle_M3/1 -> Hardware M3/1(duty_cycle)
  duty_cycle_M5/1 -> Hardware M5/1(duty_cycle)
  block_M4/1 -> Hardware M4/2(block)
  block_M3/1 -> Hardware M3/2(block)
  Hardware M4/1(v_cap) -> v_cap_M4/1
  connections:
  Hardware M5/RConn2 -- AC Load10/RConn1
  AC Load6/LConn1 -- Hardware M1/RConn1
  Hardware M1/LConn2 -- Hardware M2/LConn1
  Hardware M3/LConn2 -- Hardware M4/LConn1
  Hardware M5/RConn1 -- AC Load10/LConn1
  AC Load6/RConn1 -- Hardware M1/RConn2
  Hardware M2/RConn2 -- AC Load7/RConn1
  Hardware M2/LConn2 -- Hardware M3/LConn1
  Hardware M2/RConn1 -- AC Load7/LConn1
  Hardware M3/RConn1 -- AC Load8/LConn1
  Hardware M3/RConn2 -- AC Load8/RConn1
  Hardware M4/RConn2 -- AC Load9/RConn1
  Hardware M4/RConn1 -- AC Load9/LConn1
  Hardware M4/LConn2 -- Hardware M5/LConn1
  V1low_M1/RConn1 -- Hardware M1/LConn1
  Low_GND_M5/RConn1 -- Hardware M5/LConn2

== system MMC_phase_hackathon_consensus_PWM_JABBAR_20260927/ /Subsystem/Subsystem1 ==
  note: MMC electrical circuit connected to the modules hardware block
  note: MMC electrical circuit connected to the modules hardware block
  note: MMC electrical circuit connected to the modules hardware block
  note: MMC electrical circuit connected to the modules hardware block
  note: MMC electrical circuit connected to the modules hardware block
  duty_cycle_M1 : Inport
  block_M1 : Inport  Port=2
  duty_cycle_M2 : Inport  Port=3
  block_M2 : Inport  Port=4
  duty_cycle_M3 : Inport  Port=5
  block_M3 : Inport  Port=6
  duty_cycle_M4 : Inport  Port=7
  block_M4 : Inport  Port=8
  duty_cycle_M5 : Inport  Port=9
  block_M5 : Inport  Port=10
  AC Load{6..10} (5 alike) : spsSeriesRLCBranchLib/Series RLC Branch  LConnTagsString=__new0  RConnTagsString=__new0  BranchType=C  Resistance=R  Inductance=L_arm  SetiL0=off  InitialCurrent=0  Capacitance=C_M_extra  Setx0=on  InitialVoltage=source_V  Measurements=None
  Hardware M1 : Subsystem
  Hardware M2 : Subsystem
  Hardware M3 : Subsystem
  Hardware M4 : Subsystem
  Hardware M5 : Subsystem
  V1low_M1 : PMIOPort  Side=Left
  Low_GND_M5 : PMIOPort  Port=2  Side=Left
  i_mod_M1 : Outport
  v_cap_M1 : Outport  Port=2
  v_cap_M2 : Outport  Port=3
  v_cap_M3 : Outport  Port=4
  v_cap_M4 : Outport  Port=5
  v_cap_M5 : Outport  Port=6
  wires:
  Hardware M1/1(v_cap) -> v_cap_M1/1
  duty_cycle_M1/1 -> Hardware M1/1(duty_cycle)
  duty_cycle_M2/1 -> Hardware M2/1(duty_cycle)
  block_M5/1 -> Hardware M5/2(block)
  Hardware M3/1(v_cap) -> v_cap_M3/1
  block_M1/1 -> Hardware M1/2(block)
  Hardware M1/2(i_mod) -> i_mod_M1/1
  duty_cycle_M4/1 -> Hardware M4/1(duty_cycle)
  block_M2/1 -> Hardware M2/2(block)
  Hardware M5/1(v_cap) -> v_cap_M5/1
  Hardware M2/1(v_cap) -> v_cap_M2/1
  duty_cycle_M3/1 -> Hardware M3/1(duty_cycle)
  duty_cycle_M5/1 -> Hardware M5/1(duty_cycle)
  block_M4/1 -> Hardware M4/2(block)
  block_M3/1 -> Hardware M3/2(block)
  Hardware M4/1(v_cap) -> v_cap_M4/1
  connections:
  Hardware M5/RConn2 -- AC Load10/RConn1
  AC Load6/LConn1 -- Hardware M1/RConn1
  Hardware M1/LConn2 -- Hardware M2/LConn1
  Hardware M3/LConn2 -- Hardware M4/LConn1
  Hardware M5/RConn1 -- AC Load10/LConn1
  AC Load6/RConn1 -- Hardware M1/RConn2
  Hardware M2/RConn2 -- AC Load7/RConn1
  Hardware M2/LConn2 -- Hardware M3/LConn1
  Hardware M2/RConn1 -- AC Load7/LConn1
  Hardware M3/RConn1 -- AC Load8/LConn1
  Hardware M3/RConn2 -- AC Load8/RConn1
  Hardware M4/RConn2 -- AC Load9/RConn1
  Hardware M4/RConn1 -- AC Load9/LConn1
  Hardware M4/LConn2 -- Hardware M5/LConn1
  V1low_M1/RConn1 -- Hardware M1/LConn1
  Low_GND_M5/RConn1 -- Hardware M5/LConn2

== system MMC_phase_hackathon_consensus_PWM_JABBAR_20260927/ /Sinus Modulation + Sorting Algorithm/Subsystem1/Subsystem ==
  sm_id : Inport
  Vc_am : Inport  Port=2
  Input : Inport  Port=3
  Constant : Constant  Value=5
  MATLAB Function1 : MATLAB Function  TreatAsAtomicUnit=on
  MATLAB Function3 : MATLAB Function  TreatAsAtomicUnit=on
  gate_signal : Outport
  wires:
  [Nu_a] -> MATLAB Function3/2(m_arm)
  MATLAB Function3/1(gate_signal) -> gate_signal/1
  sm_id/1 -> MATLAB Function1/2(i), MATLAB Function3/1(sm_id)
  Input/1 -> MATLAB Function3/3(i_arm)
  Vc_am/1 -> MATLAB Function3/4(Vc_arm), MATLAB Function1/1(Vc_arm)
  MATLAB Function1/1(Vc_prev) -> MATLAB Function3/5(Vc_prev)
  MATLAB Function1/2(Vc_next) -> MATLAB Function3/6(Vc_next)
  Constant/1 -> MATLAB Function3/7(N)

== system MMC_phase_hackathon_consensus_PWM_JABBAR_20260927/ /Sinus Modulation + Sorting Algorithm/Subsystem1/Subsystem1 ==
  sm_id : Inport
  Vc_am : Inport  Port=2
  Input : Inport  Port=3
  Constant : Constant  Value=5  OutDataTypeStr=double
  MATLAB Function1 : MATLAB Function  TreatAsAtomicUnit=on
  MATLAB Function3 : MATLAB Function  TreatAsAtomicUnit=on
  gate_signal : Outport
  wires:
  MATLAB Function1/2(Vc_next) -> MATLAB Function3/6(Vc_next)
  MATLAB Function1/1(Vc_prev) -> MATLAB Function3/5(Vc_prev)
  Vc_am/1 -> MATLAB Function1/1(Vc_arm), MATLAB Function3/4(Vc_arm)
  Input/1 -> MATLAB Function3/3(i_arm)
  sm_id/1 -> MATLAB Function3/1(sm_id), MATLAB Function1/2(i)
  MATLAB Function3/1(gate_signal) -> gate_signal/1
  [Nu_a] -> MATLAB Function3/2(m_arm)
  Constant/1 -> MATLAB Function3/7(N)

== system MMC_phase_hackathon_consensus_PWM_JABBAR_20260927/ /Sinus Modulation + Sorting Algorithm/Subsystem1/Subsystem2 ==
  sm_id : Inport
  Vc_am : Inport  Port=2
  Input : Inport  Port=3
  Constant : Constant  Value=5  OutDataTypeStr=single
  MATLAB Function1 : MATLAB Function  TreatAsAtomicUnit=on
  MATLAB Function3 : MATLAB Function  TreatAsAtomicUnit=on
  gate_signal : Outport  OutDataTypeStr=double
  wires:
  [Nu_a] -> MATLAB Function3/2(m_arm)
  MATLAB Function3/1(gate_signal) -> gate_signal/1
  sm_id/1 -> MATLAB Function1/2(i), MATLAB Function3/1(sm_id)
  Input/1 -> MATLAB Function3/3(i_arm)
  Vc_am/1 -> MATLAB Function3/4(Vc_arm), MATLAB Function1/1(Vc_arm)
  MATLAB Function1/1(Vc_prev) -> MATLAB Function3/5(Vc_prev)
  MATLAB Function1/2(Vc_next) -> MATLAB Function3/6(Vc_next)
  Constant/1 -> MATLAB Function3/7(N)

== system MMC_phase_hackathon_consensus_PWM_JABBAR_20260927/ /Sinus Modulation + Sorting Algorithm/Subsystem1/Subsystem3 ==
  sm_id : Inport
  Vc_am : Inport  Port=2
  Input : Inport  Port=3
  Constant : Constant  Value=5
  MATLAB Function1 : MATLAB Function  TreatAsAtomicUnit=on
  MATLAB Function3 : MATLAB Function  TreatAsAtomicUnit=on
  gate_signal : Outport
  wires:
  MATLAB Function1/2(Vc_next) -> MATLAB Function3/6(Vc_next)
  MATLAB Function1/1(Vc_prev) -> MATLAB Function3/5(Vc_prev)
  Vc_am/1 -> MATLAB Function1/1(Vc_arm), MATLAB Function3/4(Vc_arm)
  Input/1 -> MATLAB Function3/3(i_arm)
  sm_id/1 -> MATLAB Function3/1(sm_id), MATLAB Function1/2(i)
  MATLAB Function3/1(gate_signal) -> gate_signal/1
  [Nu_a] -> MATLAB Function3/2(m_arm)
  Constant/1 -> MATLAB Function3/7(N)

== system MMC_phase_hackathon_consensus_PWM_JABBAR_20260927/ /Sinus Modulation + Sorting Algorithm/Subsystem1/Subsystem4 ==
  sm_id : Inport
  Vc_am : Inport  Port=2
  Input : Inport  Port=3
  Constant : Constant  Value=5
  MATLAB Function1 : MATLAB Function  TreatAsAtomicUnit=on
  MATLAB Function3 : MATLAB Function  TreatAsAtomicUnit=on
  gate_signal : Outport  PortDimensions=1
  wires:
  [Nu_a] -> MATLAB Function3/2(m_arm)
  MATLAB Function3/1(gate_signal) -> gate_signal/1
  sm_id/1 -> MATLAB Function1/2(i), MATLAB Function3/1(sm_id)
  Input/1 -> MATLAB Function3/3(i_arm)
  Vc_am/1 -> MATLAB Function3/4(Vc_arm), MATLAB Function1/1(Vc_arm)
  MATLAB Function1/1(Vc_prev) -> MATLAB Function3/5(Vc_prev)
  MATLAB Function1/2(Vc_next) -> MATLAB Function3/6(Vc_next)
  Constant/1 -> MATLAB Function3/7(N)

== system MMC_phase_hackathon_consensus_PWM_JABBAR_20260927/ /Sinus Modulation + Sorting Algorithm/Subsystem2/Subsystem ==
  sm_id : Inport
  Vc_am : Inport  Port=2
  Input : Inport  Port=3
  Constant : Constant  Value=5
  MATLAB Function1 : MATLAB Function  TreatAsAtomicUnit=on
  MATLAB Function3 : MATLAB Function  TreatAsAtomicUnit=on
  gate_signal : Outport
  wires:
  Constant/1 -> MATLAB Function3/7(N)
  MATLAB Function1/2(Vc_next) -> MATLAB Function3/6(Vc_next)
  MATLAB Function1/1(Vc_prev) -> MATLAB Function3/5(Vc_prev)
  Vc_am/1 -> MATLAB Function1/1(Vc_arm), MATLAB Function3/4(Vc_arm)
  Input/1 -> MATLAB Function3/3(i_arm)
  sm_id/1 -> MATLAB Function3/1(sm_id), MATLAB Function1/2(i)
  MATLAB Function3/1(gate_signal) -> gate_signal/1
  [Nl_a] -> MATLAB Function3/2(m_arm)

== system MMC_phase_hackathon_consensus_PWM_JABBAR_20260927/ /Sinus Modulation + Sorting Algorithm/Subsystem2/Subsystem1 ==
  sm_id : Inport
  Vc_am : Inport  Port=2
  Input : Inport  Port=3
  Constant : Constant  Value=5
  MATLAB Function1 : MATLAB Function  TreatAsAtomicUnit=on
  MATLAB Function3 : MATLAB Function  TreatAsAtomicUnit=on
  gate_signal : Outport
  wires:
  Constant/1 -> MATLAB Function3/7(N)
  [Nl_a] -> MATLAB Function3/2(m_arm)
  MATLAB Function3/1(gate_signal) -> gate_signal/1
  sm_id/1 -> MATLAB Function1/2(i), MATLAB Function3/1(sm_id)
  Input/1 -> MATLAB Function3/3(i_arm)
  Vc_am/1 -> MATLAB Function3/4(Vc_arm), MATLAB Function1/1(Vc_arm)
  MATLAB Function1/1(Vc_prev) -> MATLAB Function3/5(Vc_prev)
  MATLAB Function1/2(Vc_next) -> MATLAB Function3/6(Vc_next)

== system MMC_phase_hackathon_consensus_PWM_JABBAR_20260927/ /Sinus Modulation + Sorting Algorithm/Subsystem2/Subsystem2 ==
  sm_id : Inport
  Vc_am : Inport  Port=2
  Input : Inport  Port=3
  Constant : Constant  Value=5
  MATLAB Function1 : MATLAB Function  TreatAsAtomicUnit=on
  MATLAB Function3 : MATLAB Function  TreatAsAtomicUnit=on
  gate_signal : Outport
  wires:
  Constant/1 -> MATLAB Function3/7(N)
  MATLAB Function1/2(Vc_next) -> MATLAB Function3/6(Vc_next)
  MATLAB Function1/1(Vc_prev) -> MATLAB Function3/5(Vc_prev)
  Vc_am/1 -> MATLAB Function1/1(Vc_arm), MATLAB Function3/4(Vc_arm)
  Input/1 -> MATLAB Function3/3(i_arm)
  sm_id/1 -> MATLAB Function3/1(sm_id), MATLAB Function1/2(i)
  MATLAB Function3/1(gate_signal) -> gate_signal/1
  [Nl_a] -> MATLAB Function3/2(m_arm)

== system MMC_phase_hackathon_consensus_PWM_JABBAR_20260927/ /Sinus Modulation + Sorting Algorithm/Subsystem2/Subsystem3 ==
  sm_id : Inport
  Vc_am : Inport  Port=2
  Input : Inport  Port=3
  Constant : Constant  Value=5
  MATLAB Function1 : MATLAB Function  TreatAsAtomicUnit=on
  MATLAB Function3 : MATLAB Function  TreatAsAtomicUnit=on
  gate_signal : Outport
  wires:
  Constant/1 -> MATLAB Function3/7(N)
  [Nl_a] -> MATLAB Function3/2(m_arm)
  MATLAB Function3/1(gate_signal) -> gate_signal/1
  sm_id/1 -> MATLAB Function1/2(i), MATLAB Function3/1(sm_id)
  Input/1 -> MATLAB Function3/3(i_arm)
  Vc_am/1 -> MATLAB Function3/4(Vc_arm), MATLAB Function1/1(Vc_arm)
  MATLAB Function1/1(Vc_prev) -> MATLAB Function3/5(Vc_prev)
  MATLAB Function1/2(Vc_next) -> MATLAB Function3/6(Vc_next)

== system MMC_phase_hackathon_consensus_PWM_JABBAR_20260927/ /Sinus Modulation + Sorting Algorithm/Subsystem2/Subsystem4 ==
  sm_id : Inport
  Vc_am : Inport  Port=2
  Input : Inport  Port=3
  Constant : Constant  Value=5
  MATLAB Function1 : MATLAB Function  TreatAsAtomicUnit=on
  MATLAB Function3 : MATLAB Function  TreatAsAtomicUnit=on
  gate_signal : Outport
  wires:
  Constant/1 -> MATLAB Function3/7(N)
  MATLAB Function1/2(Vc_next) -> MATLAB Function3/6(Vc_next)
  MATLAB Function1/1(Vc_prev) -> MATLAB Function3/5(Vc_prev)
  Vc_am/1 -> MATLAB Function1/1(Vc_arm), MATLAB Function3/4(Vc_arm)
  Input/1 -> MATLAB Function3/3(i_arm)
  sm_id/1 -> MATLAB Function3/1(sm_id), MATLAB Function1/2(i)
  MATLAB Function3/1(gate_signal) -> gate_signal/1
  [Nl_a] -> MATLAB Function3/2(m_arm)
